simulink model "Autonomous_Vehicle_Trajectory_Tracking"  (R2024b)
settings: Solver=VariableStepAuto  StartTime=0.0  StopTime=10.0  RelTol=1e-3
values from neighbouring files (symbols this model uses):
  A = 5.0    (= 5)    [parameters.m]
  dt = 0.01    [parameters.m]
  K = 0.75    [parameters.m]
  Ks = 1.0    (= 1)    [parameters.m]
  L = 2.8    [parameters.m]
  omega = 0.05    [parameters.m]
  v_ref = 10.0    (= 10)    [parameters.m]
libraries: simulink x1
settings Model: Creator=Mohamed  LastModifiedBy=Mohamed

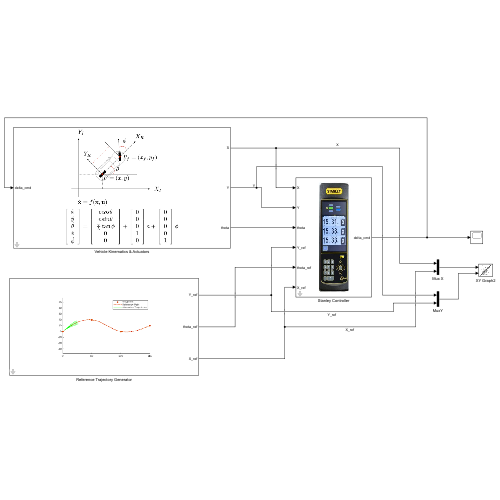
[thumbnail: Simulink's stored preview of the top-level diagram]
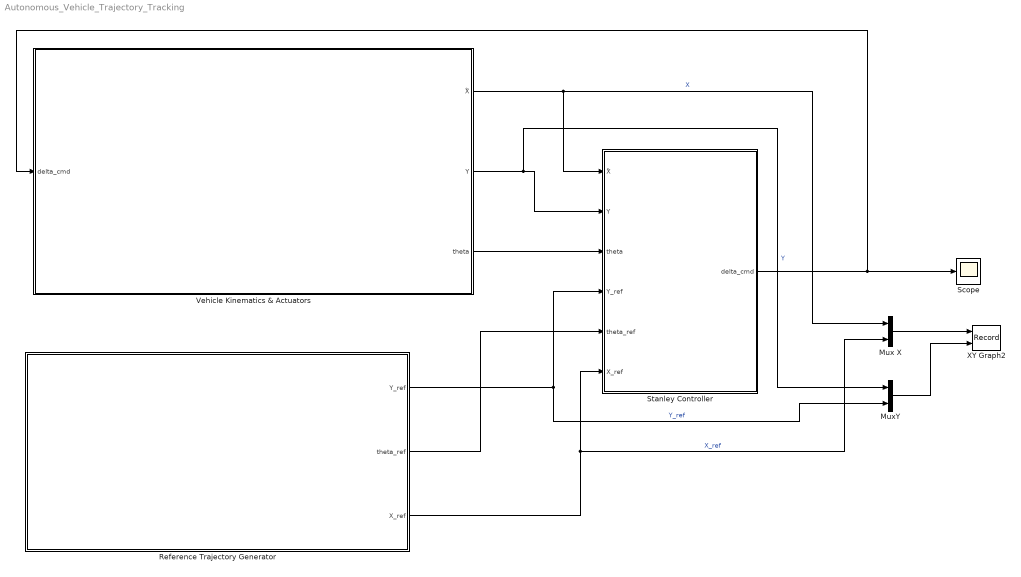
== system Autonomous_Vehicle_Trajectory_Tracking ==
  Mux X : Mux  Inputs=2
  MuxY : Mux  Inputs=2
  Reference Trajectory Generator : Subsystem  mask{A=A, omega=omega}
      mask prompts: A "Trajectory Amplitude A (m)"; omega "Trajectory Frequency omega (rad/s)"
      mask Display: image('images (1).png', [0,0,0,0,70,70]);
  Scope : Scope
  Stanley Controller : Subsystem  mask{K=-K, Ks=Ks}
      mask prompts: K "Cross-track Gain (k)"; Ks "Softening Constant (k_s)"
      mask Display: image('images.jpg');
  Vehicle Kinematics & Actuators : Subsystem  mask{L=L, v_ref=v_ref}
      mask prompts: L "Wheelbase"; v_ref "Vehicle Velocity v_ref (m/"
      mask Display: image('images.png', [0,0,0,0,70,100]);
  XY Graph2 : Record  FileSettingsInternal="{\"entries\":[{\"content\":{\"excelSettings\":{\"content\":{},\"type\":\"Streamout.ExcelSettings\"}},\"type\":\"Streamout.FileSettingStorage\",\"uuid\":\"\"}],\"packageUris\":[\"http:\\/\\/schema.mathworks.com\\/mf0\\/streamout_blocks\\/R2020a\"],\"version\":\"1.0\"}"  Layout=[1 1]  SignalsInternal="{\"entries\":[{\"content\":{\"signals\":[{\"content\":{\"blockPath\":[],\"dimensions\":[2],\"domain\":\"\",\"hasChildren\":true,\"lineColor\":\"#fe330a\",\"lineWidth\":2,\"port\":1,\"sid\":[\"\"],\"signalID\":1,\"signalName\":\"Mux X\"},\"type\":\"RecordBlkView.Signal\",\"uuid\":\"\"},{\"content\":{\"blockPath\":[],\"channel\":[1],\"dimensions\":[2],\"domain\":\"\",\"lineColor\":\"#139fff\",\"lineWidth\":2,\"parentID\":1,\"plots\":[ 1 ],\"port\":1,\"sid\":[\"\"],\"signalID\":2,\"signalName\":\"Mux X\"},\"type\":\"RecordBlkView.Signal\",\"uuid\":\"\"},{\"content\":{\"blockPath\":[],\"dimensions\":[2],\"domain\":\"\",\"hasChildren\":true,\"lineColor\":\"#0072bd\",\"lineWidth\":2,\"port\":2,\"sid\":[\"\"],\"signalID\":3,\"signalName\":\"MuxY\"},\"type\":\"RecordBlkView.Signal\",\"uuid\":\"\"},{\"content\":{\"blockPath\":[],\"channel\":[1],\"dimensions\":[2],\"domain\":\"\",\"lineColor\":\"#b746ff\",\"lineWidth\":2,\"parentID\":3,\"plots\":[ 1 ],\"port\":2,\"sid\":[\"\"],\"signalID\":4,\"signalName\":\"MuxY\"},\"type\":\"RecordBlkView.Signal\",\"uuid\":\"\"},{\"content\":{\"blockPath\":[],\"channel\":[2],\"dimensions\":[2],\"domain\":\"\",\"lineColor\":\"#64d413\",\"lineWidth\":2,\"parentID\":1,\"plots\":[ 1 ],\"port\":1,\"sid\":[\"\"],\"signalID\":5,\"signalName\":\"Mux X\"},\"type\":\"RecordBlkView.Signal\",\"uuid\":\"\"},{\"content\":{\"blockPath\":[],\"channel\":[2],\"dimensions\":[2],\"domain\":\"\",\"lineColor\":\"#ff13a6\",\"lineWidth\":2,\"parentID\":3,\"plots\":[ 1 ],\"port\":2,\"sid\":[\"\"],\"signalID\":6,\"signalName\":\"MuxY\"},\"type\":\"RecordBlkView.Signal\",\"uuid\":\"\"}]},\"type\":\"RecordBlkView.InputSignals\",\"uuid\":\"\"}],\"packageUris\":[\"http:\\/\\/schema.mathworks.com\\/mf0\\/streamout_blocks\\/R2020a\"],\"version\":\"1.0\"}"  VisualizationBindings="{\"xyplotplugin\":{\"info\":[{\"series\":[{\"bindingParametersList\":[{\"parameter\":\"X-Axis\",\"signalID\":2,\"signalName\":\"Mux X(1)\"},{\"parameter\":\"Y-Axis\",\"signalID\":4,\"signalName\":\"MuxY(1)\"}],\"seriesID\":0},{\"bindingParametersList\":[{\"parameter\":\"X-Axis\",\"signalID\":5,\"signalName\":\"Mux X(2)\"},{\"parameter\":\"Y-Axis\",\"signalID\":6,\"signalName\":\"MuxY(2)\"}],\"seriesID\":1},{\"bindingParametersList\":[{\"parameter\":\"X-Axis\",\"signalID\":6,\"signalName\":\"MuxY(2)\"}],\"seriesID\":2}],\"subplotID\":1}]}}"  CompatibilityTag=XY
  wires:
  Vehicle Kinematics & Actuators/1(ْX) -> Mux X/1, Stanley Controller/1(ْX)  "X"
  Vehicle Kinematics & Actuators/2(Y) -> MuxY/1, Stanley Controller/2(Y)  "Y"
  Vehicle Kinematics & Actuators/3(theta) -> Stanley Controller/3(theta)
  Reference Trajectory Generator/1(Y_ref) -> MuxY/2, Stanley Controller/4(Y_ref)  "Y_ref"
  Reference Trajectory Generator/2(theta_ref) -> Stanley Controller/5(theta_ref)
  Reference Trajectory Generator/3(X_ref) -> Mux X/2, Stanley Controller/6(X_ref)  "X_ref"
  Stanley Controller/1(delta_cmd) -> Scope/1, Vehicle Kinematics & Actuators/1(delta_cmd)
  Mux X/1 -> XY Graph2/1
  MuxY/1 -> XY Graph2/2

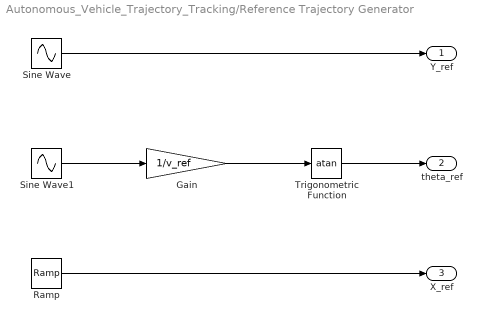
== system Autonomous_Vehicle_Trajectory_Tracking/Reference Trajectory Generator ==
  Gain : Gain  Gain=1/v_ref
  Ramp : simulink/Sources/Ramp  slope=v_ref  start=0  InitialOutput=0
  Sine Wave : Sin  Amplitude=5  Frequency=.05  SampleTime=0
  Sine Wave1 : Sin  Amplitude=0.25  Frequency=.05  Phase=pi/2  SampleTime=dt
  Trigonometric Function : Trigonometry  Operator=atan
  Y_ref : Outport
  theta_ref : Outport  Port=2
  X_ref : Outport  Port=3
  wires:
  Gain/1 -> Trigonometric Function/1
  Sine Wave1/1 -> Gain/1
  Sine Wave/1 -> Y_ref/1
  Trigonometric Function/1 -> theta_ref/1
  Ramp/1 -> X_ref/1

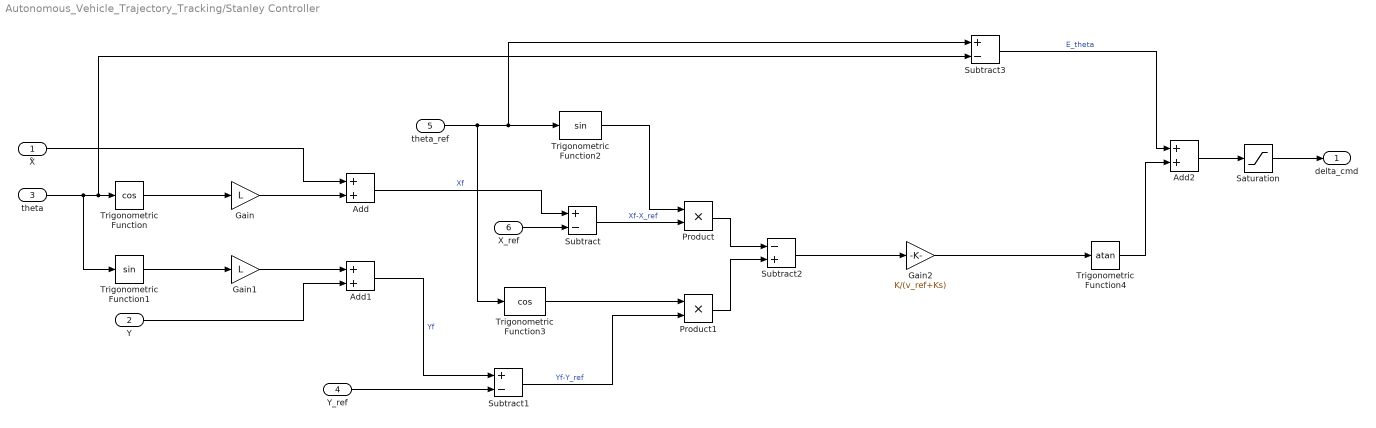
== system Autonomous_Vehicle_Trajectory_Tracking/Stanley Controller ==
  ْX : Inport
  Y : Inport  Port=2
  theta : Inport  Port=3
  Y_ref : Inport  Port=4
  theta_ref : Inport  Port=5
  X_ref : Inport  Port=6
  Add : Sum
  Add1 : Sum
  Add2 : Sum
  Gain : Gain  Gain=L
  Gain1 : Gain  Gain=L
  Gain2 : Gain  Gain=K/(v_ref+Ks)
  Product : Product
  Product1 : Product
  Saturation : Saturate  UpperLimit=0.5236  LowerLimit=-0.5236
  Subtract : Sum  Inputs=+-
  Subtract1 : Sum  Inputs=+-
  Subtract2 : Sum  Inputs=-+
  Subtract3 : Sum  Inputs=+-
  Trigonometric Function : Trigonometry  Operator=cos
  Trigonometric Function1 : Trigonometry
  Trigonometric Function2 : Trigonometry
  Trigonometric Function3 : Trigonometry  Operator=cos
  Trigonometric Function4 : Trigonometry  Operator=atan
  delta_cmd : Outport
  wires:
  theta/1 -> Trigonometric Function1/1, Subtract3/2, Trigonometric Function/1
  Trigonometric Function/1 -> Gain/1
  ْX/1 -> Add/1
  Gain/1 -> Add/2
  Trigonometric Function1/1 -> Gain1/1
  Gain1/1 -> Add1/1
  Y/1 -> Add1/2
  Add/1 -> Subtract/1  "Xf"
  X_ref/1 -> Subtract/2
  theta_ref/1 -> Subtract3/1, Trigonometric Function2/1, Trigonometric Function3/1
  Trigonometric Function2/1 -> Product/1
  Subtract/1 -> Product/2  "Xf-X_ref"
  Y_ref/1 -> Subtract1/2
  Add1/1 -> Subtract1/1  "Yf"
  Trigonometric Function3/1 -> Product1/1
  Subtract1/1 -> Product1/2  "Yf-Y_ref"
  Product/1 -> Subtract2/1
  Product1/1 -> Subtract2/2
  Subtract2/1 -> Gain2/1
  Gain2/1 -> Trigonometric Function4/1
  Subtract3/1 -> Add2/1  "E_theta"
  Trigonometric Function4/1 -> Add2/2
  Add2/1 -> Saturation/1
  Saturation/1 -> delta_cmd/1

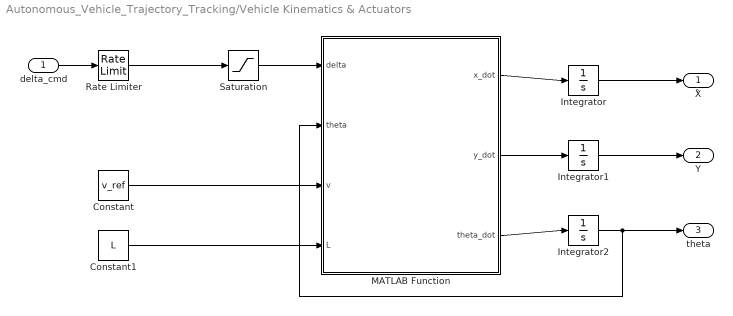
== system Autonomous_Vehicle_Trajectory_Tracking/Vehicle Kinematics & Actuators ==
  delta_cmd : Inport
  Constant : Constant  Value=v_ref
  Constant1 : Constant  Value=L
  Integrator : Integrator
  Integrator1 : Integrator
  Integrator2 : Integrator
  MATLAB Function : MATLAB Function  TreatAsAtomicUnit=on
  Rate Limiter : RateLimiter  RisingSlewLimit=1.047  FallingSlewLimit=-1.047  SampleTimeMode=inherited
  Saturation : Saturate  UpperLimit=0.5236  LowerLimit=-0.5236
  ْX : Outport
  Y : Outport  Port=2
  theta : Outport  Port=3
  wires:
  Constant1/1 -> MATLAB Function/4(L)
  Integrator2/1 -> theta/1, MATLAB Function/2(theta)
  Saturation/1 -> MATLAB Function/1(delta)
  Rate Limiter/1 -> Saturation/1
  Constant/1 -> MATLAB Function/3(v)
  MATLAB Function/1(x_dot) -> Integrator/1
  MATLAB Function/2(y_dot) -> Integrator1/1
  MATLAB Function/3(theta_dot) -> Integrator2/1
  Integrator1/1 -> Y/1
  delta_cmd/1 -> Rate Limiter/1
  Integrator/1 -> ْX/1

== matlab function Autonomous_Vehicle_Trajectory_Tracking/Vehicle Kinematics & Actuators/MATLAB Function ==
  data: delta input; x_dot output; theta input; v input; L input; y_dot output; theta_dot output
function [x_dot, y_dot, theta_dot] = vehicle_kinematics(delta, theta, v, L)
    % Bicycle Kinematic Model Equations
    x_dot     = v * cos(theta);
    y_dot     = v * sin(theta);
    theta_dot = (v / L) * tan(delta);
end
